simulink model "Histogram_equilization_"  (R2023b)
settings: Solver=VariableStepAuto  StartTime=0.0  StopTime=10.0  RelTol=1e-3
libraries: visionhdlio x4, dspvision x1
settings Model: Creator=snmz4  LastModifiedBy=snmz4

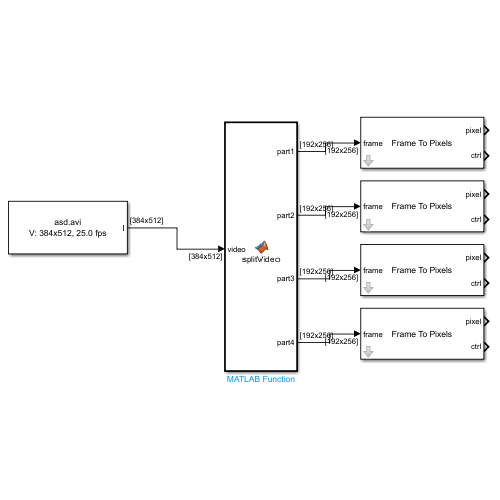
[thumbnail: Simulink's stored preview of the top-level diagram]
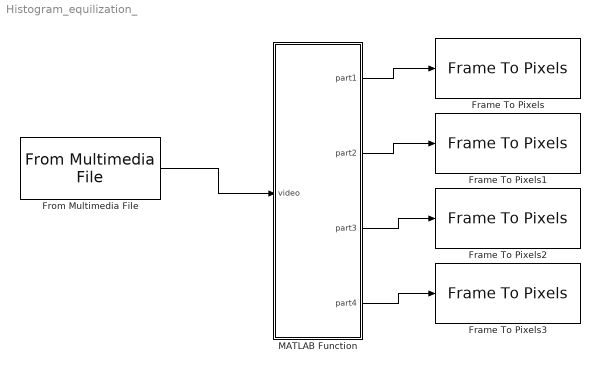
== system Histogram_equilization_ ==
  Frame To Pixels : visionhdlio/Frame To Pixels  NumComponents=1  NumPixels=8  VideoFormat=1080p  ActivePixelsPerLine=1920  ActiveVideoLines=1080  TotalPixelsPerLine=2200  TotalVideoLines=1125  StartingActiveLine=42  FrontPorch=88  SampleTime=0  VideoFormatCache=1080p  ActivePixelsPerLineCache=32  ActiveVideoLinesCache=18  TotalPixelsPerLineCache=42  TotalVideoLinesCache=28  StartingActiveLineCache=6  FrontPorchCache=5
  Frame To Pixels1 : visionhdlio/Frame To Pixels  NumComponents=1  NumPixels=8  VideoFormat=1080p  ActivePixelsPerLine=1920  ActiveVideoLines=1080  TotalPixelsPerLine=2200  TotalVideoLines=1125  StartingActiveLine=42  FrontPorch=88  SampleTime=0  VideoFormatCache=1080p  ActivePixelsPerLineCache=32  ActiveVideoLinesCache=18  TotalPixelsPerLineCache=42  TotalVideoLinesCache=28  StartingActiveLineCache=6  FrontPorchCache=5
  Frame To Pixels2 : visionhdlio/Frame To Pixels  NumComponents=1  NumPixels=8  VideoFormat=240p  ActivePixelsPerLine=320  ActiveVideoLines=240  TotalPixelsPerLine=402  TotalVideoLines=324  StartingActiveLine=1  FrontPorch=44  SampleTime=0  VideoFormatCache=240p  ActivePixelsPerLineCache=32  ActiveVideoLinesCache=18  TotalPixelsPerLineCache=42  TotalVideoLinesCache=28  StartingActiveLineCache=6  FrontPorchCache=5
  Frame To Pixels3 : visionhdlio/Frame To Pixels  NumComponents=1  NumPixels=8  VideoFormat=1080p  ActivePixelsPerLine=1920  ActiveVideoLines=1080  TotalPixelsPerLine=2200  TotalVideoLines=1125  StartingActiveLine=42  FrontPorch=88  SampleTime=0  VideoFormatCache=1080p  ActivePixelsPerLineCache=32  ActiveVideoLinesCache=18  TotalPixelsPerLineCache=42  TotalVideoLinesCache=28  StartingActiveLineCache=6  FrontPorchCache=5
  From Multimedia File : dspvision/From Multimedia File  inputFilename=C:\Users\snmz4\Downloads\asd.avi  readRange=[1 Inf]  loop=on  numPlays=inf  outputStreams=Video only  videoDataType=double  audioDataType=int16  inheritSampleTime=on  userDefinedSampleTime=1/30  noAudioOutput=off  isIntensityVideo=off  fourcc=Intensity  colorVideoFormat=One multidimensional signal  outputEOF=off  dataOrg=Column-major  audioFrameSize=1024  computeAudioFrameSize=off  outSamplingMode=Sample based
      settings: LibrarySourceBlock=visionsources/From Multimedia File
  MATLAB Function : MATLAB Function  TreatAsAtomicUnit=on
  wires:
  MATLAB Function/1(part1) -> Frame To Pixels/1
  MATLAB Function/2(part2) -> Frame To Pixels1/1
  MATLAB Function/3(part3) -> Frame To Pixels2/1
  MATLAB Function/4(part4) -> Frame To Pixels3/1
  From Multimedia File/1 -> MATLAB Function/1(video)

== matlab function Histogram_equilization_/MATLAB Function ==
  data: video input; part1 output; part2 output; part3 output; part4 output
function [part1, part2, part3, part4] = splitVideo(video)
    % Girişlerin boyutlarını ve türlerini al
    [rows, cols, ~] = size(video);
    
    % Görüntüyü dört eşit parçaya böl
    rows_half = floor(rows / 2);
    cols_half = floor(cols / 2);
    
    % Girişin ilk yarısını parçalara ata
    part1 = video(1:rows_half, 1:cols_half, :);
    part2 = video(1:rows_half, cols_half+1:end, :);
    part3 = video(rows_half+1:end, 1:cols_half, :);
    part4 = video(rows_half+1:end, cols_half+1:end, :);
end
